simulink model "PMLSM_PI_FOC_Float_Baseline"  (R2026b)
settings: Solver=FixedStepDiscrete  StopTime=M1A_StopTime_s  FixedStep=Ts_Plant
InitFcn:
  | m1a_require_float_init(bdroot);
values from neighbouring files (symbols this model uses):
  Alignment_Enable = 0    [init_PMLSM_PI_FOC_Float_Baseline.m]
  Hold_Ticks = 30000    [init_PMLSM_PI_FOC_Float_Baseline.m]
  Host_AutoStart_EN = 1    [init_PMLSM_PI_FOC_Float_Baseline.m]
  Host_Close_Loop_EN = 1    [init_PMLSM_PI_FOC_Float_Baseline.m]
  Host_Id_A = 0    [init_PMLSM_PI_FOC_Float_Baseline.m]
  Host_Iq_A = 0    [init_PMLSM_PI_FOC_Float_Baseline.m]
  Host_Iq_Test_Mode = 0    [init_PMLSM_PI_FOC_Float_Baseline.m]
  Host_Load_N = 0    [init_PMLSM_PI_FOC_Float_Baseline.m]
  Host_Move_Request = 0    [init_PMLSM_PI_FOC_Float_Baseline.m]
  Host_PI_Reset_EN = 0    [init_PMLSM_PI_FOC_Float_Baseline.m]
  Host_Position_Loop_EN = 1    [init_PMLSM_PI_FOC_Float_Baseline.m]
  Host_PWM_EN = 1    [init_PMLSM_PI_FOC_Float_Baseline.m]
  Host_Ready_Ticks = 5    [init_PMLSM_PI_FOC_Float_Baseline.m]
  Host_Replay_EN = 0    [init_PMLSM_PI_FOC_Float_Baseline.m]
  Host_Speed_mmps = 0    [init_PMLSM_PI_FOC_Float_Baseline.m]
  Host_Speed_Ramp_s = 0.1    [init_PMLSM_PI_FOC_Float_Baseline.m]
  Host_Start_s = 0.05    [init_PMLSM_PI_FOC_Float_Baseline.m]
  Host_Target_mm = 10    [init_PMLSM_PI_FOC_Float_Baseline.m]
  Host_Traj_Amax = 100    [init_PMLSM_PI_FOC_Float_Baseline.m]
  Host_Traj_Jmax = 1000    [init_PMLSM_PI_FOC_Float_Baseline.m]
  Host_Traj_Vmax = 10    [init_PMLSM_PI_FOC_Float_Baseline.m]
  Id_Init_Step = Id_Init_Target/Ramp_Ticks    (= 5e-05)    [init_PMLSM_PI_FOC_Float_Baseline.m]
  Id_Init_Target = 0.5    [init_PMLSM_PI_FOC_Float_Baseline.m]
  Id_Release_Ramp_Ticks = 2000    [init_PMLSM_PI_FOC_Float_Baseline.m]
  Init_Reset = 0    [init_PMLSM_PI_FOC_Float_Baseline.m]
  Init_Start = 0    [init_PMLSM_PI_FOC_Float_Baseline.m]
  Iq_int_limit = 0.5    [init_PMLSM_PI_FOC_Float_Baseline.m]
  Kaw_d = Tuning_Gains.Kaw_d    [init_PMLSM_PI_FOC_Float_Baseline.m]
  Kaw_q = Tuning_Gains.Kaw_q    [init_PMLSM_PI_FOC_Float_Baseline.m]
  Kaw_s = Tuning_Gains.Kaw_s    [init_PMLSM_PI_FOC_Float_Baseline.m]
  Ki_ACR = Tuning_Gains.Ki_ACR    [init_PMLSM_PI_FOC_Float_Baseline.m]
  Ki_ASR = Tuning_Gains.Ki_ASR    [init_PMLSM_PI_FOC_Float_Baseline.m]
  Kp_ACR = Tuning_Gains.Kp_ACR    [init_PMLSM_PI_FOC_Float_Baseline.m]
  Kp_ASR = Tuning_Gains.Kp_ASR    [init_PMLSM_PI_FOC_Float_Baseline.m]
  Kp_pos = Tuning_Gains.Kp_pos    [init_PMLSM_PI_FOC_Float_Baseline.m]
  M1A_PWM_Update_Delay_s = T_pwm/2    (= 5e-05)    [init_PMLSM_PI_FOC_Float_Baseline.m]
  PMLSM_Bv_N_per_mps = 0    [init_PMLSM_PI_FOC_Float_Baseline.m]
  PMLSM_deadtime_current_eps_A = 1e-4    (= 0.0001)    [init_PMLSM_PI_FOC_Float_Baseline.m]
  PMLSM_deadtime_ratio = PMLSM_deadtime_s/T_pwm    (= 0.01)    [init_PMLSM_PI_FOC_Float_Baseline.m]
  PMLSM_Fc_N = 0    [init_PMLSM_PI_FOC_Float_Baseline.m]
  PMLSM_Kf_peak_N_per_Apeak = 31.4/sqrt(2)    [init_PMLSM_PI_FOC_Float_Baseline.m]
  PMLSM_Ld_H = 1.745e-3    (= 0.001745)    [init_PMLSM_PI_FOC_Float_Baseline.m]
  PMLSM_Lq_H = PMLSM_Ld_H    (= 0.001745)    [init_PMLSM_PI_FOC_Float_Baseline.m]
  PMLSM_M_kg = 0.91    [init_PMLSM_PI_FOC_Float_Baseline.m]
  PMLSM_psi_f_Wb = 0.141    [init_PMLSM_PI_FOC_Float_Baseline.m]
  PMLSM_Rs_ohm = 2.37    [init_PMLSM_PI_FOC_Float_Baseline.m]
  PMLSM_tau_NN_m = 0.06    [init_PMLSM_PI_FOC_Float_Baseline.m]
  PMLSM_theta_offset_rad = 0    [init_PMLSM_PI_FOC_Float_Baseline.m]
  PMLSM_Ts_s = Ts_Plant    (= 1e-06)    [init_PMLSM_PI_FOC_Float_Baseline.m]
  PMLSM_v_eps_mps = 1e-3    (= 0.001)    [init_PMLSM_PI_FOC_Float_Baseline.m]
  Pos_deadband = 0.02    [init_PMLSM_PI_FOC_Float_Baseline.m]
  Ramp_Ticks = 10000    [init_PMLSM_PI_FOC_Float_Baseline.m]
  Simulation_Travel_Fault = 0    [init_PMLSM_PI_FOC_Float_Baseline.m]
  Speed_loop_Iq_Limit = 1    [init_PMLSM_PI_FOC_Float_Baseline.m]
  T_pwm = 1e-4    (= 0.0001)    [init_PMLSM_PI_FOC_Float_Baseline.m]
  Tau_e_mm = PMLSM_tau_NN_m*1000    (= 60)    [init_PMLSM_PI_FOC_Float_Baseline.m]
  theta_align_const = 0    [init_PMLSM_PI_FOC_Float_Baseline.m]
  Theta_Offset_Fine = 0    [init_PMLSM_PI_FOC_Float_Baseline.m]
  Ts = Ts_ACR    (= 0.0001)    [init_PMLSM_PI_FOC_Float_Baseline.m]
  Ts_ACR = T_pwm    (= 0.0001)    [init_PMLSM_PI_FOC_Float_Baseline.m]
  Ts_ASR = 10*Ts_ACR    (= 0.001)    [init_PMLSM_PI_FOC_Float_Baseline.m]
  Ts_Plant = 1e-6    (= 1e-06)    [init_PMLSM_PI_FOC_Float_Baseline.m]
  Ts_POS = 10*Ts_ASR    (= 0.01)    [init_PMLSM_PI_FOC_Float_Baseline.m]
  Udc = 48    [init_PMLSM_PI_FOC_Float_Baseline.m]
  v_ff_eps = 0.5    [init_PMLSM_PI_FOC_Float_Baseline.m]
  v_over_eps = 3    [init_PMLSM_PI_FOC_Float_Baseline.m]
  V_pos_max_mmps = 20    [init_PMLSM_PI_FOC_Float_Baseline.m]
  v_ref_max = 20    [init_PMLSM_PI_FOC_Float_Baseline.m]
  v_ref_set_step_dn = v_ref_set_rate_dn*Ts_ACR    (= 0.005)    [init_PMLSM_PI_FOC_Float_Baseline.m]
  v_ref_set_step_up = v_ref_set_rate_up*Ts_ACR    (= 0.005)    [init_PMLSM_PI_FOC_Float_Baseline.m]
  v_ref_zero_eps = 0    [init_PMLSM_PI_FOC_Float_Baseline.m]
undefined symbols (not defined in the file or in its folder): DiscIntNeverNeededParam, Iq_fric_run, Iq_fric_start, v_stick_off, v_stick_on
libraries: simulink x7, mcbeeMathTransformLib x2
(part 2 of 2)

== system PMLSM_PI_FOC_Float_Baseline/Control_Task_10kHz/Speed_Loop/friction_compensation ==
  note: if start_mode == 1
      | 	iq_fric_mag = Iq_fric_start;
      | else
      | 	iq_fric_mag = Iq_fric_run;
      |
      | if ff_enable
      | 	iq_ff = iq_fric_mag * sign(v_ref);
      |  else
      | 	iq_ff = 0;
  v_ref : Inport
  abs_v_ref : Inport  Port=2
  abs_v_mmps : Inport  Port=3
  e_v : Inport  Port=4
  Compare To Constant1 : simulink/Logic and Bit Operations/Compare To Constant  relop=>  const=-v_over_eps  OutDataTypeStr=boolean
  Compare To Constant2 : simulink/Logic and Bit Operations/Compare To Constant  relop=>  const=v_ff_eps  OutDataTypeStr=boolean
  Constant1 : Constant  Value=Iq_fric_start
  Constant5 : Constant  Value=0
  Constant6 : Constant  Value=Iq_fric_run
  Gain : Gain  Gain=-1
  Logical Operator : Logic  AllPortsSameDT=off  OutDataTypeStr=boolean
  Product : Product
  Product1 : Product
  Product2 : Product
  Relay : Relay  OnSwitchValue=-v_stick_on  OffSwitchValue=-v_stick_off
  Sign : Signum
  Sign1 : Signum
  Switch : Switch  Criteria=u2 > Threshold  Threshold=0.5  SaturateOnIntegerOverflow=off  InputSameDT=off
  Switch2 : Switch  Criteria=u2 > Threshold  Threshold=0.5  SaturateOnIntegerOverflow=off  InputSameDT=off
  iq_ff : Outport
  wires:
  v_ref/1 -> Sign/1, Sign1/1
  Sign/1 -> Product2/1, Product/1
  Constant5/1 -> Switch2/3
  Constant6/1 -> Product/2
  abs_v_ref/1 -> Compare To Constant2/1
  Switch2/1 -> iq_ff/1  "iq_ff"
  Switch/1 -> Switch2/1
  Product/1 -> Switch/3
  Sign1/1 -> Product1/1
  Constant1/1 -> Product1/2
  Product1/1 -> Switch/1
  e_v/1 -> Product2/2
  Product2/1 -> Compare To Constant1/1
  Compare To Constant2/1 -> Logical Operator/1
  Compare To Constant1/1 -> Logical Operator/2
  Logical Operator/1 -> Switch2/2  "ff_enable"
  abs_v_mmps/1 -> Gain/1
  Relay/1 -> Switch/2  "fric_start_mode"
  Gain/1 -> Relay/1

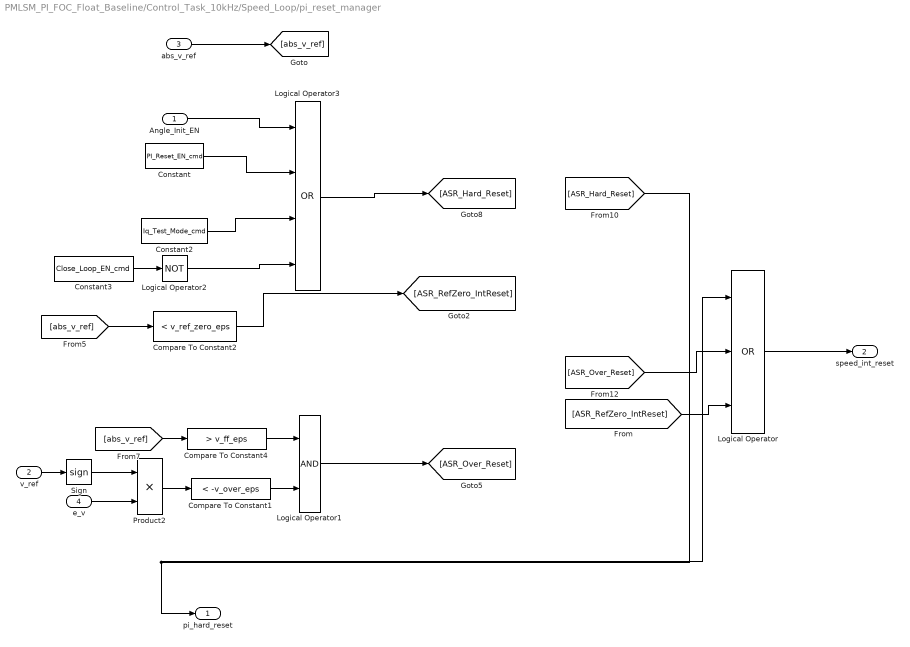
== system PMLSM_PI_FOC_Float_Baseline/Control_Task_10kHz/Speed_Loop/pi_reset_manager ==
  Angle_Init_EN : Inport
  v_ref : Inport  Port=2
  abs_v_ref : Inport  Port=3
  e_v : Inport  Port=4
  Compare To Constant1 : simulink/Logic and Bit Operations/Compare To Constant  relop=<  const=-v_over_eps  OutDataTypeStr=boolean
  Compare To Constant2 : simulink/Logic and Bit Operations/Compare To Constant  relop=<  const=v_ref_zero_eps  OutDataTypeStr=boolean
  Compare To Constant4 : simulink/Logic and Bit Operations/Compare To Constant  relop=>  const=v_ff_eps  OutDataTypeStr=boolean
  Constant : DataStoreRead  DataStoreName=PI_Reset_EN_cmd  IndexOptions=Index vector (dialog)  Indices=1  OutputSizes=1
  Constant2 : DataStoreRead  DataStoreName=Iq_Test_Mode_cmd  IndexOptions=Index vector (dialog)  Indices=1  OutputSizes=1
  Constant3 : DataStoreRead  DataStoreName=Close_Loop_EN_cmd  IndexOptions=Index vector (dialog)  Indices=1  OutputSizes=1
  Logical Operator : Logic  Operator=OR  Inputs=3  AllPortsSameDT=off  OutDataTypeStr=boolean
  Logical Operator1 : Logic  AllPortsSameDT=off  OutDataTypeStr=boolean
  Logical Operator2 : Logic  Operator=NOT  AllPortsSameDT=off  OutDataTypeStr=boolean
  Logical Operator3 : Logic  Operator=OR  Inputs=4  AllPortsSameDT=off  OutDataTypeStr=boolean
  Product2 : Product
  Sign : Signum
  pi_hard_reset : Outport
  speed_int_reset : Outport  Port=2
  wires:
  Compare To Constant2/1 -> [ASR_RefZero_IntReset]
  [abs_v_ref] -> Compare To Constant2/1
  [abs_v_ref] -> Compare To Constant4/1
  e_v/1 -> Product2/2
  Sign/1 -> Product2/1
  Product2/1 -> Compare To Constant1/1
  Compare To Constant1/1 -> Logical Operator1/2
  Compare To Constant4/1 -> Logical Operator1/1
  v_ref/1 -> Sign/1
  abs_v_ref/1 -> [abs_v_ref]
  Logical Operator1/1 -> [ASR_Over_Reset]
  [ASR_RefZero_IntReset] -> Logical Operator/3
  Logical Operator/1 -> speed_int_reset/1
  [ASR_Over_Reset] -> Logical Operator/2
  [ASR_Hard_Reset] -> pi_hard_reset/1, Logical Operator/1
  Logical Operator3/1 -> [ASR_Hard_Reset]
  Angle_Init_EN/1 -> Logical Operator3/1
  Logical Operator2/1 -> Logical Operator3/4
  Constant2/1 -> Logical Operator3/3
  Constant3/1 -> Logical Operator2/1
  Constant/1 -> Logical Operator3/2

== system PMLSM_PI_FOC_Float_Baseline/Inverter_DeadTime/DeadTime_Voltage_Model/Phase_A_DeadTime ==
  duty : Inport
  i_phase : Inport  Port=2
  deadtime_ratio : Inport  Port=3
  vdc : Inport  Port=4
  d_sat : Saturate  UpperLimit=1  LowerLimit=0
  d_sum : Sum  Inputs=+-
  delta_d : Product  Inputs=**
  i_deadzone : DeadZone  LowerValue=-PMLSM_deadtime_current_eps_A  UpperValue=PMLSM_deadtime_current_eps_A
  sign_i : Signum
  v0_eff_calc : Product
  v0_eff : Outport
  wires:
  v0_eff_calc/1 -> v0_eff/1  "inv_a_v0_eff"
  vdc/1 -> v0_eff_calc/2
  d_sat/1 -> v0_eff_calc/1  "inv_a_d_eff"
  i_phase/1 -> i_deadzone/1
  i_deadzone/1 -> sign_i/1
  sign_i/1 -> delta_d/1  "inv_a_sign_i"
  deadtime_ratio/1 -> delta_d/2
  delta_d/1 -> d_sum/2  "inv_a_delta_d"
  d_sum/1 -> d_sat/1  "inv_a_d_unsat"
  duty/1 -> d_sum/1

== system PMLSM_PI_FOC_Float_Baseline/Inverter_DeadTime/DeadTime_Voltage_Model/Phase_B_DeadTime ==
  duty : Inport
  i_phase : Inport  Port=2
  deadtime_ratio : Inport  Port=3
  vdc : Inport  Port=4
  d_sat : Saturate  UpperLimit=1  LowerLimit=0
  d_sum : Sum  Inputs=+-
  delta_d : Product  Inputs=**
  i_deadzone : DeadZone  LowerValue=-PMLSM_deadtime_current_eps_A  UpperValue=PMLSM_deadtime_current_eps_A
  sign_i : Signum
  v0_eff_calc : Product
  v0_eff : Outport
  wires:
  v0_eff_calc/1 -> v0_eff/1  "inv_b_v0_eff"
  vdc/1 -> v0_eff_calc/2
  d_sat/1 -> v0_eff_calc/1  "inv_b_d_eff"
  i_phase/1 -> i_deadzone/1
  i_deadzone/1 -> sign_i/1
  sign_i/1 -> delta_d/1  "inv_b_sign_i"
  deadtime_ratio/1 -> delta_d/2
  delta_d/1 -> d_sum/2  "inv_b_delta_d"
  d_sum/1 -> d_sat/1  "inv_b_d_unsat"
  duty/1 -> d_sum/1

== system PMLSM_PI_FOC_Float_Baseline/Inverter_DeadTime/DeadTime_Voltage_Model/Phase_C_DeadTime ==
  duty : Inport
  i_phase : Inport  Port=2
  deadtime_ratio : Inport  Port=3
  vdc : Inport  Port=4
  d_sat : Saturate  UpperLimit=1  LowerLimit=0
  d_sum : Sum  Inputs=+-
  delta_d : Product  Inputs=**
  i_deadzone : DeadZone  LowerValue=-PMLSM_deadtime_current_eps_A  UpperValue=PMLSM_deadtime_current_eps_A
  sign_i : Signum
  v0_eff_calc : Product
  v0_eff : Outport
  wires:
  v0_eff_calc/1 -> v0_eff/1  "inv_c_v0_eff"
  vdc/1 -> v0_eff_calc/2
  d_sat/1 -> v0_eff_calc/1  "inv_c_d_eff"
  i_phase/1 -> i_deadzone/1
  i_deadzone/1 -> sign_i/1
  sign_i/1 -> delta_d/1  "inv_c_sign_i"
  deadtime_ratio/1 -> delta_d/2
  delta_d/1 -> d_sum/2  "inv_c_delta_d"
  d_sum/1 -> d_sat/1  "inv_c_d_unsat"
  duty/1 -> d_sum/1

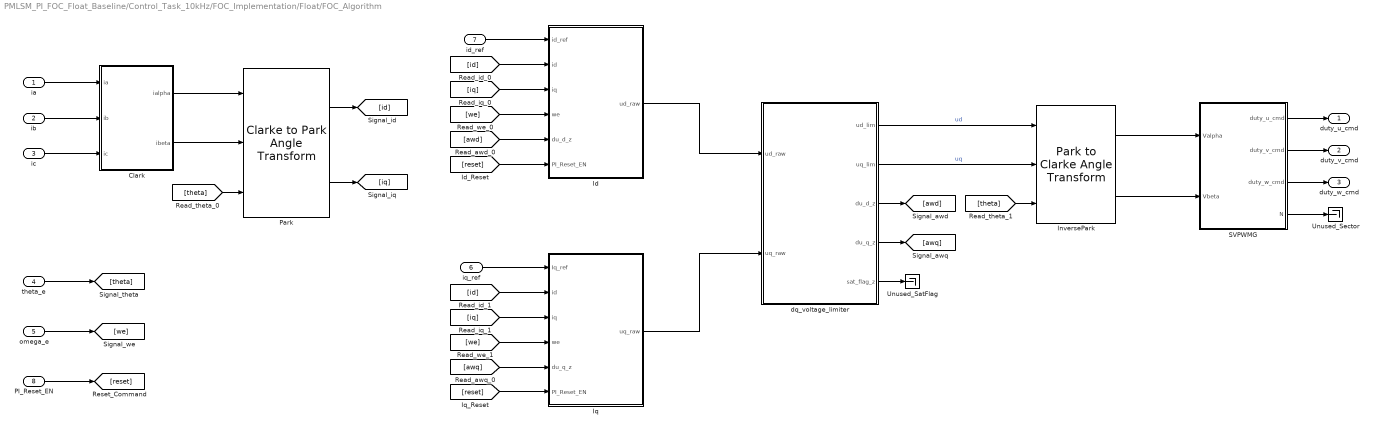
== system PMLSM_PI_FOC_Float_Baseline/Control_Task_10kHz/FOC_Implementation/Float/FOC_Algorithm ==
  ia : Inport
  ib : Inport  Port=2
  ic : Inport  Port=3
  theta_e : Inport  Port=4
  omega_e : Inport  Port=5
  iq_ref : Inport  Port=6
  id_ref : Inport  Port=7
  PI_Reset_EN : Inport  Port=8
  Clark : Subsystem  TreatAsAtomicUnit=on  RTWFcnName=Clack_Fun
      settings: RTWFcnNameOpts=User specified
  Id : Subsystem  TreatAsAtomicUnit=on  RTWFcnName=Id_Fun
      settings: RTWFcnNameOpts=User specified
  InversePark : mcbeeMathTransformLib/Park to Clarke Angle Transform  AxisAlignment=D-axis  UseWithEmbedded=on  PhaseInput=Two inputs  ThetaInput=Electrical position  AngleInput=Radians  N_points=1024
      settings: LibrarySourceBlock=mcbhdllib/Controls/Math Transforms/Inverse Park Transform
  Iq : Subsystem  TreatAsAtomicUnit=on  RTWFcnName=Iq_Fun
      settings: RTWFcnNameOpts=User specified
  Park : mcbeeMathTransformLib/Clarke to Park Angle Transform  AxisAlignment=D-axis  UseWithEmbedded=on  PhaseInput=Two inputs  ThetaInput=Electrical position  AngleInput=Radians  N_points=1024
      settings: LibrarySourceBlock=mcblib/Controls/Math Transforms/Park Transform
  SVPWMG : Subsystem  TreatAsAtomicUnit=on  RTWFcnName=SVPWM_Gen_Fun
      settings: RTWFcnNameOpts=User specified
  Unused_SatFlag : Terminator
  Unused_Sector : Terminator
  dq_voltage_limiter : Subsystem
  duty_u_cmd : Outport
  duty_v_cmd : Outport  Port=2
  duty_w_cmd : Outport  Port=3
  wires:
  SVPWMG/4("N ") -> Unused_Sector/1
  SVPWMG/3(duty_w_cmd) -> duty_w_cmd/1
  SVPWMG/2(duty_v_cmd) -> duty_v_cmd/1
  SVPWMG/1(duty_u_cmd) -> duty_u_cmd/1
  ic/1 -> Clark/3(ic)
  ib/1 -> Clark/2(ib)
  ia/1 -> Clark/1(ia)
  [theta] -> InversePark/3
  [theta] -> Park/3
  Clark/1(ialpha) -> Park/1
  Clark/2(ibeta) -> Park/2
  theta_e/1 -> [theta]
  Park/1 -> [id]
  Park/2 -> [iq]
  omega_e/1 -> [we]
  dq_voltage_limiter/3(du_d_z) -> [awd]
  dq_voltage_limiter/4(du_q_z) -> [awq]
  dq_voltage_limiter/5(sat_flag_z) -> Unused_SatFlag/1
  dq_voltage_limiter/1(ud_lim) -> InversePark/1  "ud"
  dq_voltage_limiter/2(uq_lim) -> InversePark/2  "uq"
  InversePark/1 -> SVPWMG/1(Valpha)
  InversePark/2 -> SVPWMG/2(Vbeta)
  [reset] -> Iq/6(PI_Reset_EN)
  [reset] -> Id/6(PI_Reset_EN)
  id_ref/1 -> Id/1(id_ref)
  PI_Reset_EN/1 -> [reset]
  Iq/1(uq_raw) -> dq_voltage_limiter/2(uq_raw)
  Id/1(ud_raw) -> dq_voltage_limiter/1(ud_raw)
  iq_ref/1 -> Iq/1(Iq_ref)
  [id] -> Id/2(id)
  [id] -> Iq/2(id)
  [iq] -> Id/3(iq)
  [iq] -> Iq/3(iq)
  [we] -> Id/4(we)
  [we] -> Iq/4(we)
  [awd] -> Id/5(du_d_z)
  [awq] -> Iq/5(du_q_z)

== system PMLSM_PI_FOC_Float_Baseline/Control_Task_10kHz/FOC_Implementation/Float/FOC_Algorithm/Clark ==
  note: alpha=(A-0.5*(B+C))*2/3
      | Beta=sqrt(3)/2*(B-C)*2/3
  ia : Inport
  ib : Inport  Port=2
  ic : Inport  Port=3
  Add : Sum  Inputs=+--
  Add1 : Sum  Inputs=+-
  Gain : Gain  Gain=0.5
  Gain1 : Gain  Gain=0.5
  Gain2 : Gain  Gain=2/3
  Gain3 : Gain  Gain=1/sqrt(3)
  ialpha : Outport
  ibeta : Outport  Port=2
  wires:
  Gain/1 -> Add/2
  Gain2/1 -> ialpha/1  "ialf"
  Add/1 -> Gain2/1
  Gain3/1 -> ibeta/1  "ibeta"
  ic/1 -> Gain1/1, Add1/2
  Add1/1 -> Gain3/1
  ib/1 -> Gain/1, Add1/1
  ia/1 -> Add/1
  Gain1/1 -> Add/3

== system PMLSM_PI_FOC_Float_Baseline/Control_Task_10kHz/FOC_Implementation/Float/FOC_Algorithm/Id ==
  note: 起到使能时初始化一下的作用
  id_ref : Inport
  id : Inport  Port=2
  iq : Inport  Port=3
  we : Inport  Port=4
  du_d_z : Inport  Port=5
  PI_Reset_EN : Inport  Port=6
  " " : Gain  Gain=Ki_ACR*Ts_ACR
  "  " : Gain  Gain=Kp_ACR
  Add1 : Sum
  Add2 : Sum  Inputs=++-
  Constant1 : Constant  Value=PMLSM_Lq_H
  Gain : Gain  Gain=Kaw_d
  Product : Product
  Product1 : Product
  Reset_Integral : Switch  Criteria=u2 > Threshold  Threshold=0.5  SaturateOnIntegerOverflow=off  InputSameDT=off
  Reset_Output : Switch  Criteria=u2 > Threshold  Threshold=0.5  SaturateOnIntegerOverflow=off  InputSameDT=off
  Reset_Zero : Constant  Value=0
  Sum : Sum  Inputs=|+-
  Sum1 : Sum  Inputs=|+-
  x_d_z : UnitDelay  SampleTime=-1
  ud_raw : Outport
  wires:
  [du_d_z] -> Gain/1
  [x_d_next] -> x_d_z/1
  du_d_z/1 -> [du_d_z]
  "  "/1 -> Add1/1
  Constant1/1 -> Product/2
  Product/1 -> Product1/1
  we/1 -> Product1/2
  Sum/1 -> "  "/1, " "/1
  id/1 -> Sum/2
  id_ref/1 -> Sum/1
  iq/1 -> Product/1
  Reset_Output/1 -> ud_raw/1
  Reset_Integral/1 -> [x_d_next]
  PI_Reset_EN/1 -> Reset_Output/2, Reset_Integral/2
  Reset_Zero/1 -> Reset_Output/1, Reset_Integral/1
  Add2/1 -> Reset_Integral/3  "x_d_next"
  Sum1/1 -> Reset_Output/3
  " "/1 -> Add2/2  "KiTs_q * e_d"
  Gain/1 -> Add2/3  "u_d,aw"
  x_d_z/1 -> Add2/1, Add1/2
  Add1/1 -> Sum1/1
  Product1/1 -> Sum1/2  "解耦项"

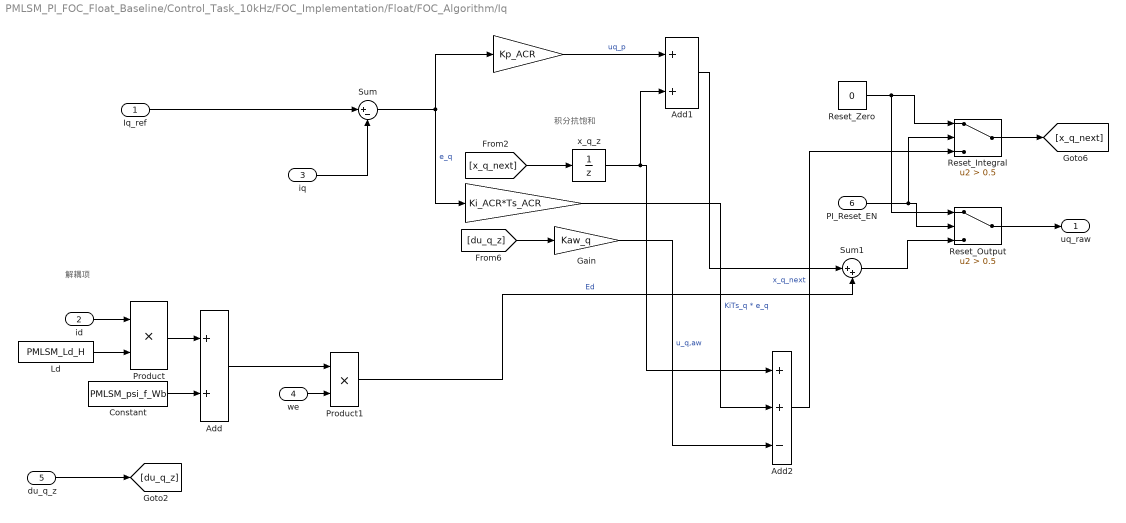
== system PMLSM_PI_FOC_Float_Baseline/Control_Task_10kHz/FOC_Implementation/Float/FOC_Algorithm/Iq ==
  note: 积分抗饱和
  note: 解耦项
  Iq_ref : Inport
  id : Inport  Port=2
  iq : Inport  Port=3
  we : Inport  Port=4
  du_q_z : Inport  Port=5
  PI_Reset_EN : Inport  Port=6
  " " : Gain  Gain=Ki_ACR*Ts_ACR
  "  " : Gain  Gain=Kp_ACR
  Add : Sum
  Add1 : Sum
  Add2 : Sum  Inputs=++-
  Constant : Constant  Value=PMLSM_psi_f_Wb
  Gain : Gain  Gain=Kaw_q
  Ld : Constant  Value=PMLSM_Ld_H
  Product : Product
  Product1 : Product
  Reset_Integral : Switch  Criteria=u2 > Threshold  Threshold=0.5  SaturateOnIntegerOverflow=off  InputSameDT=off
  Reset_Output : Switch  Criteria=u2 > Threshold  Threshold=0.5  SaturateOnIntegerOverflow=off  InputSameDT=off
  Reset_Zero : Constant  Value=0
  Sum : Sum  Inputs=|+-
  Sum1 : Sum  Inputs=|++
  x_q_z : UnitDelay  SampleTime=-1
  uq_raw : Outport
  wires:
  Iq_ref/1 -> Sum/1
  [x_q_next] -> x_q_z/1
  [du_q_z] -> Gain/1
  du_q_z/1 -> [du_q_z]
  "  "/1 -> Add1/1  "uq_p"
  Sum/1 -> " "/1, "  "/1  "e_q"
  Add/1 -> Product1/1
  Constant/1 -> Add/2
  Product/1 -> Add/1
  Ld/1 -> Product/2
  id/1 -> Product/1
  iq/1 -> Sum/2
  we/1 -> Product1/2
  Reset_Output/1 -> uq_raw/1
  Reset_Integral/1 -> [x_q_next]
  PI_Reset_EN/1 -> Reset_Output/2, Reset_Integral/2
  Reset_Zero/1 -> Reset_Output/1, Reset_Integral/1
  Add2/1 -> Reset_Integral/3  "x_q_next"
  Sum1/1 -> Reset_Output/3
  x_q_z/1 -> Add2/1, Add1/2
  " "/1 -> Add2/2  "KiTs_q * e_q"
  Gain/1 -> Add2/3  "u_q,aw"
  Add1/1 -> Sum1/1
  Product1/1 -> Sum1/2  "Ed"

== system PMLSM_PI_FOC_Float_Baseline/Control_Task_10kHz/FOC_Implementation/Float/FOC_Algorithm/SVPWMG ==
  Valpha : Inport
  Vbeta : Inport  Port=2
  Duty Calculate : Subsystem  TreatAsAtomicUnit=on  RTWFcnName=Duty_Caculate_Fun
      settings: RTWFcnNameOpts=User specified
  Sector Caculate : Subsystem  TreatAsAtomicUnit=on  RTWFcnName=Sector_Caculate_Fun
      settings: RTWFcnNameOpts=User specified
  T1T2 Calculate : Subsystem  TreatAsAtomicUnit=on  RTWFcnName=T1T2Caculate_Fun
      settings: RTWFcnNameOpts=User specified
  Udc : Constant  Value=Udc
  XYZ Calculate : Subsystem  TreatAsAtomicUnit=on  RTWFcnName=XYZ_Caculate_Fun
      settings: RTWFcnNameOpts=User specified
  duty_u_cmd : Outport
  duty_v_cmd : Outport  Port=2
  duty_w_cmd : Outport  Port=3
  "N " : Outport  Port=4
  wires:
  Duty Calculate/3(Duty_W) -> duty_w_cmd/1
  Duty Calculate/2(Duty_V) -> duty_v_cmd/1
  Duty Calculate/1(Duty_U) -> duty_u_cmd/1
  XYZ Calculate/3(Z) -> T1T2 Calculate/4(Z)
  XYZ Calculate/2(Y) -> T1T2 Calculate/3(Y)
  XYZ Calculate/1(X) -> T1T2 Calculate/2(X)
  Udc/1 -> XYZ Calculate/3(Udc)
  Sector Caculate/1("N ") -> T1T2 Calculate/1(N), Duty Calculate/1(N), "N "/1
  T1T2 Calculate/2(T2) -> Duty Calculate/3(T2)
  Valpha/1 -> XYZ Calculate/1(Ualpha), Sector Caculate/1(Ualpha)
  T1T2 Calculate/1(T1) -> Duty Calculate/2(T1)
  Vbeta/1 -> XYZ Calculate/2(Ubeta), Sector Caculate/2(Ubeta)

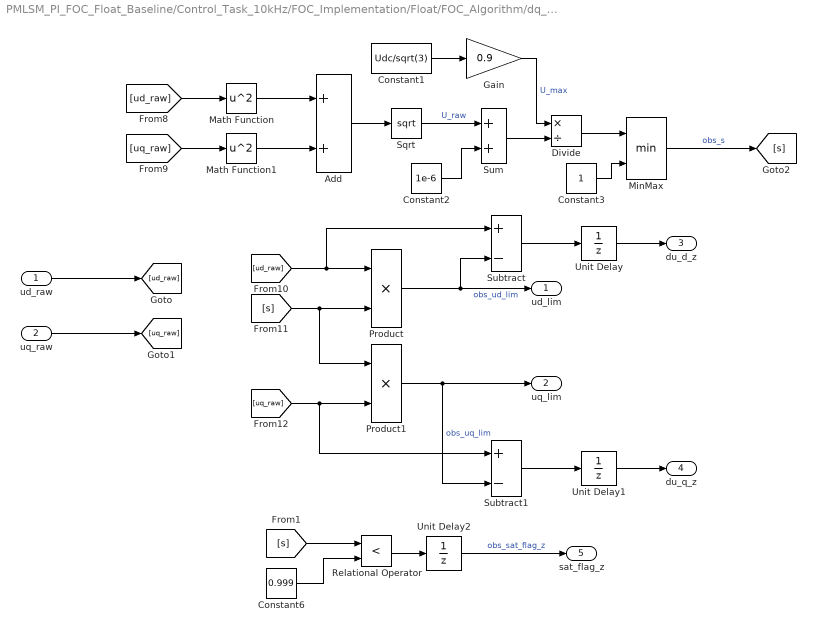
== system PMLSM_PI_FOC_Float_Baseline/Control_Task_10kHz/FOC_Implementation/Float/FOC_Algorithm/dq_voltage_limiter ==
  ud_raw : Inport
  uq_raw : Inport  Port=2
  Add : Sum
  Constant1 : Constant  Value=Udc/sqrt(3)  OutDataTypeStr=double
  Constant2 : Constant  Value=1e-6  OutDataTypeStr=double
  Constant3 : Constant  OutDataTypeStr=double
  Constant6 : Constant  Value=0.999
  Divide : Product  Inputs=*/  OutDataTypeStr=double
  Gain : Gain  Gain=0.9  OutDataTypeStr=double
  Math Function : Math  Operator=square
  Math Function1 : Math  Operator=square
  MinMax : MinMax  Inputs=2
  Product : Product
  Product1 : Product  OutDataTypeStr=double
  Relational Operator : RelationalOperator  Operator=<  OutDataTypeStr=boolean  RndMeth=Simplest  InputSameDT=off
  Sqrt : Sqrt
  Subtract : Sum  Inputs=+-
  Subtract1 : Sum  Inputs=+-
  Sum : Sum
  Unit Delay : UnitDelay  SampleTime=-1
  Unit Delay1 : UnitDelay  SampleTime=-1
  Unit Delay2 : UnitDelay  SampleTime=-1
  ud_lim : Outport
  uq_lim : Outport  Port=2
  du_d_z : Outport  Port=3
  du_q_z : Outport  Port=4
  sat_flag_z : Outport  Port=5
  wires:
  Unit Delay2/1 -> sat_flag_z/1  "obs_sat_flag_z"
  Relational Operator/1 -> Unit Delay2/1
  [s] -> Relational Operator/1
  Constant6/1 -> Relational Operator/2
  Unit Delay1/1 -> du_q_z/1
  Unit Delay/1 -> du_d_z/1
  uq_raw/1 -> [uq_raw]
  ud_raw/1 -> [ud_raw]
  Subtract1/1 -> Unit Delay1/1
  Subtract/1 -> Unit Delay/1
  [uq_raw] -> Product1/2, Subtract1/1
  Product/1 -> ud_lim/1, Subtract/2  "obs_ud_lim"
  [ud_raw] -> Product/1, Subtract/1
  [s] -> Product/2, Product1/1
  Product1/1 -> Subtract1/2, uq_lim/1  "obs_uq_lim"
  MinMax/1 -> [s]  "obs_s"
  [ud_raw] -> Math Function/1
  [uq_raw] -> Math Function1/1
  Math Function/1 -> Add/1
  Math Function1/1 -> Add/2
  Sqrt/1 -> Sum/1  "U_raw"
  Gain/1 -> Divide/1  "U_max"
  Divide/1 -> MinMax/1
  Constant1/1 -> Gain/1
  Add/1 -> Sqrt/1
  Constant3/1 -> MinMax/2
  Constant2/1 -> Sum/2
  Sum/1 -> Divide/2

== system PMLSM_PI_FOC_Float_Baseline/Control_Task_10kHz/FOC_Implementation/Float/FOC_Algorithm/SVPWMG/Duty Calculate ==
  N : Inport
  T1 : Inport  Port=2
  T2 : Inport  Port=3
  Constant : Constant  Value=Ts
  Fcn : Fcn  Expr=(u[3]-u[1]-u[2])/4
  Fcn1 : Fcn  Expr=(u[3]+u[1]-u[2])/4
  Fcn2 : Fcn  Expr=(u[3]+u[2]+u[1])/4
  Gain : Gain  Gain=-2/T_pwm
  Gain1 : Gain  Gain=-2/T_pwm
  Gain1_UpperDuty : Bias  Bias=1  SaturateOnIntegerOverflow=off
  Gain2 : Gain  Gain=-2/T_pwm
  Gain2_UpperDuty : Bias  Bias=1  SaturateOnIntegerOverflow=off
  Gain_UpperDuty : Bias  Bias=1  SaturateOnIntegerOverflow=off
  Multiport Switch : MultiPortSwitch  Inputs=6  SaturateOnIntegerOverflow=off  InputSameDT=off
  Multiport Switch1 : MultiPortSwitch  Inputs=6  SaturateOnIntegerOverflow=off  InputSameDT=off
  Multiport Switch2 : MultiPortSwitch  Inputs=6  SaturateOnIntegerOverflow=off  InputSameDT=off
  Mux : Mux  Inputs=3
  Duty_U : Outport
  Duty_V : Outport  Port=2
  Duty_W : Outport  Port=3
  wires:
  N/1 -> Multiport Switch/1, Multiport Switch1/1, Multiport Switch2/1
  Fcn2/1 -> Multiport Switch2/4, Multiport Switch2/2, Multiport Switch1/7, Multiport Switch1/3, Multiport Switch/6, Multiport Switch/5
  Fcn1/1 -> Multiport Switch/2, Multiport Switch/7, Multiport Switch1/4, Multiport Switch2/6, Multiport Switch2/3, Multiport Switch1/5
  Fcn/1 -> Multiport Switch1/2, Multiport Switch2/7, Multiport Switch2/5, Multiport Switch1/6, Multiport Switch/4, Multiport Switch/3
  Multiport Switch/1 -> Gain/1
  Multiport Switch1/1 -> Gain1/1
  Multiport Switch2/1 -> Gain2/1
  T1/1 -> Mux/1
  T2/1 -> Mux/2
  Constant/1 -> Mux/3
  Mux/1 -> Fcn1/1, Fcn/1, Fcn2/1
  Gain/1 -> Gain_UpperDuty/1  "DutyU"
  Gain_UpperDuty/1 -> Duty_U/1
  Gain1/1 -> Gain1_UpperDuty/1  "DutyV"
  Gain1_UpperDuty/1 -> Duty_V/1
  Gain2/1 -> Gain2_UpperDuty/1  "DutyW"
  Gain2_UpperDuty/1 -> Duty_W/1

== system PMLSM_PI_FOC_Float_Baseline/Control_Task_10kHz/FOC_Implementation/Float/FOC_Algorithm/SVPWMG/Sector Caculate ==
  Ualpha : Inport
  Ubeta : Inport  Port=2
  B0 : Fcn  Expr=u[2]
  B1 : Fcn  Expr=u[1]*0.866-0.5*u[2]
  B2 : Fcn  Expr=-u[1]*0.866-u[2]*0.5
  Constant : Constant
  Constant1 : Constant  Value=0
  Mux : Mux  Inputs=2
  Mux1 : Mux  Inputs=3
  N : Fcn  Expr=4*u[3]+2*u[2]+u[1]
  Switch : Switch  Criteria=u2 > Threshold  SaturateOnIntegerOverflow=off  InputSameDT=off
  Switch1 : Switch  SaturateOnIntegerOverflow=off  InputSameDT=off
  Switch2 : Switch  Criteria=u2 > Threshold  SaturateOnIntegerOverflow=off  InputSameDT=off
  "N " : Outport  VectorParamsAs1DForOutWhenUnconnected=off
  wires:
  N/1 -> "N "/1  "N"
  Mux1/1 -> N/1
  Switch1/1 -> Mux1/2
  Constant1/1 -> Switch2/3, Switch1/3, Switch/3
  Constant/1 -> Switch1/1, Switch2/1, Switch/1
  B2/1 -> Switch2/2
  B1/1 -> Switch1/2
  B0/1 -> Switch/2
  Mux/1 -> B0/1, B1/1, B2/1
  Ubeta/1 -> Mux/2
  Ualpha/1 -> Mux/1
  Switch/1 -> Mux1/1
  Switch2/1 -> Mux1/3

== system PMLSM_PI_FOC_Float_Baseline/Control_Task_10kHz/FOC_Implementation/Float/FOC_Algorithm/SVPWMG/T1T2 Calculate ==
  N : Inport
  X : Inport  Port=2
  Y : Inport  Port=3
  Z : Inport  Port=4
  Constant : Constant  Value=Ts
  Fcn : Fcn  Expr=u(3)-u(2)-u(1)
  Fcn1 : Fcn  Expr=u(1)*u(3)/(u(1)+u(2))
  Fcn2 : Fcn  Expr=u(2)*u(3)/(u(1)+u(2))
  Gain : Gain  Gain=-1
  Gain1 : Gain  Gain=-1
  Gain2 : Gain  Gain=-1
  Multiport Switch : MultiPortSwitch  Inputs=6  SaturateOnIntegerOverflow=off  InputSameDT=off
  Multiport Switch1 : MultiPortSwitch  Inputs=6  SaturateOnIntegerOverflow=off  InputSameDT=off
  Mux : Mux  Inputs=3
  Switch : Switch  SaturateOnIntegerOverflow=off  InputSameDT=off
  Switch1 : Switch  Criteria=u2 > Threshold  SaturateOnIntegerOverflow=off  InputSameDT=off
  T1 : Outport  VectorParamsAs1DForOutWhenUnconnected=off
  T2 : Outport  Port=2  VectorParamsAs1DForOutWhenUnconnected=off
  wires:
  Gain1/1 -> Multiport Switch/7, Multiport Switch1/6
  Gain2/1 -> Multiport Switch1/7, Multiport Switch/4
  Gain/1 -> Multiport Switch/5, Multiport Switch1/3
  X/1 -> Multiport Switch1/4, Multiport Switch/6, Gain/1
  Z/1 -> Gain2/1, Multiport Switch/2, Multiport Switch1/5
  Y/1 -> Gain1/1, Multiport Switch1/2, Multiport Switch/3
  N/1 -> Multiport Switch1/1, Multiport Switch/1
  Multiport Switch1/1 -> Mux/2, Switch1/1
  Multiport Switch/1 -> Mux/1, Switch/1
  Mux/1 -> Fcn2/1, Fcn/1, Fcn1/1
  Fcn/1 -> Switch1/2, Switch/2
  Fcn1/1 -> Switch/3
  Fcn2/1 -> Switch1/3
  Switch/1 -> T1/1  "T1"
  Switch1/1 -> T2/1  "T2"
  Constant/1 -> Mux/3

== system PMLSM_PI_FOC_Float_Baseline/Control_Task_10kHz/FOC_Implementation/Float/FOC_Algorithm/SVPWMG/XYZ Calculate ==
  Ualpha : Inport
  Ubeta : Inport  Port=2
  Udc : Inport  Port=3
  Add : Sum
  Add1 : Sum  Inputs=+-
  Constant1 : Constant  Value=Ts
  Gain : Gain  Gain=3/2
  Gain1 : Gain  Gain=1.7321
  Gain2 : Gain  Gain=0.866
  Math Function : Math  Operator=reciprocal
  Product{,1..3} (4 alike) : Product
  X : Outport
  Y : Outport  Port=2
  Z : Outport  Port=3
  wires:
  Constant1/1 -> Product/1
  Product3/1 -> Y/1  "Y"
  Product2/1 -> Z/1  "Z"
  Add1/1 -> Product2/1
  Add/1 -> Product3/1
  Product1/1 -> X/1  "X"
  Gain/1 -> Add/2, Add1/2
  Gain2/1 -> Add1/1, Add/1
  Product/1 -> Product1/2, Product3/2, Product2/2
  Gain1/1 -> Product1/1
  Ubeta/1 -> Gain1/1, Gain2/1
  Math Function/1 -> Product/2
  Udc/1 -> Math Function/1
  Ualpha/1 -> Gain/1

== stateflow chart PMLSM_PI_FOC_Float_Baseline/Alignment_Task_10kHz/Enabled_Original_MIL/Angle_Init ==
  state IDLE
    entry:
    Angle_Init_EN   = 0;
    Init_Done       = 0;
    id_init_ref     = 0;
    Init_State_Num  = 0;
  note: 固定电角度，缓慢建立 d 轴电流。
  note: 保持固定电角度，让动子吸附稳定。
  state RAMP_ID
    entry:
    Angle_Init_EN   = 1;
    Init_Done       = 0;
    id_init_ref     = 0;
    Init_State_Num  = 1;
    during:
    Angle_Init_EN = 1;
    Init_Done     = 0;
    id_init_ref = id_init_ref + Id_Init_Step;
    if (id_init_ref > Id_Init_Target)
    id_init_ref = Id_Init_Target;
    end
  state HOLD_ALIGN
    entry:
    Angle_Init_EN   = 1;
    Init_Done       = 0;
    id_init_ref     = Id_Init_Target;
    Init_State_Num  = 2;
    during:
    Angle_Init_EN = 1;
    Init_Done     = 0;
    id_init_ref   = Id_Init_Target;
  state RAMP_DOWN_ID
    entry:
    Angle_Init_EN   = 1;
    Init_Done       = 0;
    id_init_ref     = Id_Init_Target;
    Init_State_Num  = 3;
    during:
    Angle_Init_EN = 1;
    Init_Done     = 0;
    id_init_ref = id_init_ref - Id_Init_Target/Id_Release_Ramp_Ticks;
    if (id_init_ref < 0)
    id_init_ref = 0;
    end
    Theta_Offset_auto = theta_offset_mem;
  state DONE
    entry:
    Angle_Init_EN   = 0;
    Init_Done       = 1;
    id_init_ref     = 0;
    Init_State_Num  = 4;
    during:
    Angle_Init_EN = 0;
    Init_Done = 1;
    id_init_ref = 0;
    Init_State_Num = 4;
    Theta_Offset_auto = theta_offset_mem;
  HOLD_ALIGN -> IDLE [order 1] : [Init_Reset > 0.5 || travel_fault_latch > 0.5]
  RAMP_ID -> IDLE [order 1] : [Init_Reset > 0.5 || travel_fault_latch > 0.5]
  (default) -> IDLE
  IDLE -> RAMP_ID : [Init_Start > 0.5 && Init_Reset < 0.5 && travel_fault_latch < 0.5]
  RAMP_ID -> HOLD_ALIGN [order 2] : [after(Ramp_Ticks, tick)]
  RAMP_DOWN_ID -> IDLE [order 2] : [Init_Reset > 0.5 || travel_fault_latch > 0.5]
  DONE -> IDLE : [Init_Reset > 0.5 || travel_fault_latch > 0.5]
  HOLD_ALIGN -> RAMP_DOWN_ID [order 2] : [after(Hold_Ticks, tick)]
      | {x_align_mm_latch = x_mm;
      | theta_offset_mem = mod(theta_align_const - 2*pi*x_align_mm_latch/Tau_e_mm, 2*pi);
      | Theta_Offset_auto = theta_offset_mem;}
  RAMP_DOWN_ID -> DONE [order 1] : [after(Id_Release_Ramp_Ticks, tick)]
  data: Init_Start input; Init_Reset input; travel_fault_latch input; Init_Done output; Init_State_Num output; theta_align_const parameter; Tau_e_mm parameter; Id_Init_Target parameter; Ramp_Ticks parameter; Hold_Ticks parameter; Id_Init_Step parameter; id_init_ref output; Angle_Init_EN output; x_mm input; Theta_Offset_auto output; x_align_mm_latch output; theta_offset_mem local; Id_Release_Ramp_Ticks parameter

== matlab function PMLSM_PI_FOC_Float_Baseline/Simple_Host/Host_Core ==
  settings: updateMethod=DISCRETE  sampleTime=Ts_ACR
  data: t input; u input; replay input; x_actual_mm input; alignment_enabled input; alignment_ready input; x_ref_mm output; vdc output; load_N output; Close_Loop_EN output; Position_Loop_EN output; PWM_EN output; v_ref_cmd output; id_ref_cmd output; iq_test_mode output; iq_test_ref output; PI_Reset_EN output; Host_Start_s parameter; Udc parameter; Host_Load_N parameter; Host_Traj_Vmax parameter; Host_Traj_Amax parameter; Host_Traj_Jmax parameter; Host_Speed_Ramp_s parameter; target_accepted_mm output; move_busy output; in_position output; command_status output; segment_start_mm output; segment_start_s output; trajectory_done output; move_ready output; accepted_count output; rejected_count output; segment_id output; command_received_s output; move_interrupted output; Ts_ACR parameter; Ts_POS parameter; Pos_deadband parameter; Host_Ready_Ticks parameter; Host_AutoStart_EN parameter; trajectory_config output
function [x_ref_mm,vdc,load_N,Close_Loop_EN,Position_Loop_EN,PWM_EN,v_ref_cmd,id_ref_cmd,iq_test_mode,iq_test_ref,PI_Reset_EN,target_accepted_mm,move_busy,in_position,command_status,segment_start_mm,segment_start_s,trajectory_done,move_ready,accepted_count,rejected_count,segment_id,command_received_s,move_interrupted,trajectory_config]=Simple_Host(t,u,replay,x_actual_mm,alignment_enabled,alignment_ready,Host_Start_s,Udc,Host_Load_N,Host_Traj_Vmax,Host_Traj_Amax,Host_Traj_Jmax,Host_Speed_Ramp_s,Ts_ACR, Ts_POS, Pos_deadband, Host_Ready_Ticks, Host_AutoStart_EN)
persistent move_state
if isempty(move_state),move_state=zeros(1,22);end
v_ref_cmd=u(2);id_ref_cmd=u(3);iq_test_mode=u(4);iq_test_ref=u(5);Position_Loop_EN=u(6);Close_Loop_EN=u(7);PWM_EN=u(8);PI_Reset_EN=u(9);
if u(10)~=0,v_ref_cmd=replay(1);PWM_EN=replay(2);PI_Reset_EN=replay(3);end
cfg=[Ts_ACR Ts_POS Host_Start_s Host_Traj_Vmax Host_Traj_Amax Host_Traj_Jmax Host_Speed_Ramp_s Pos_deadband Host_Ready_Ticks Host_AutoStart_EN];
[move_state,x_ref_mm,o]=pmlsm_point_move_step(move_state,t,x_actual_mm,u(1),u(11),Position_Loop_EN~=0 && Close_Loop_EN~=0 && iq_test_mode==0,PWM_EN,PI_Reset_EN,alignment_enabled,alignment_ready,cfg);
target_accepted_mm=o(1);move_busy=o(2);in_position=o(3);command_status=o(4);segment_start_mm=o(5);segment_start_s=o(6);trajectory_done=o(7);move_ready=o(8);accepted_count=o(9);rejected_count=o(10);segment_id=o(11);command_received_s=o(12);move_interrupted=o(13);
if alignment_enabled~=0 && alignment_ready==0
 Position_Loop_EN=0;Close_Loop_EN=0;iq_test_mode=1;iq_test_ref=0;
end
trajectory_config=[Host_Traj_Vmax Host_Traj_Amax Host_Traj_Jmax Host_Speed_Ramp_s Ts_ACR];
vdc=Udc;load_N=Host_Load_N;
end
